simulink model "Lab5_14102026"  (R2019a)
settings: Solver=VariableStepAuto  StartTime=0.0  StopTime=2  RelTol=1e-3  EnableMultiTasking=on
libraries: dspsigops x1
settings Model: Creator=CSE  LastModifiedBy=Admin
settings DataIOCC: ReturnWorkspaceOutputs=off
settings OptimizationCC: LifeSpan=inf
settings DebuggingCC: SFUnexpectedBacktrackingDiag=warning  SFNoUnconditionalDefaultTransitionDiag=warning  ArithmeticOperatorsInVariantConditions=warning
settings SFSimCC: SimUseLocalCustomCode=off
settings RTWCC: RTWUseLocalCustomCode=off
settings CodeAppCC: StateflowObjectComments=on
settings GRTTargetCC: TargetLangStandard=C89/C90 (ANSI)  GeneratePreprocessorConditionals=Disable all
settings ConfigComp: CovMetricSettings=dw  CovHtmlReporting=on  CovSaveCumulativeToWorkspaceVar=on  CovSaveSingleToWorkspaceVar=on  CovExternalEMLEnable=off

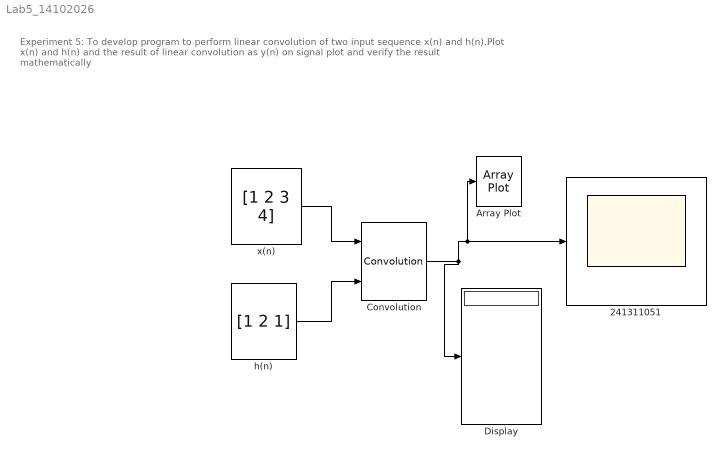
== system Lab5_14102026 ==
  note: Experiment 5: To develop program to perform linear convolution of two input sequence x(n) and h(n).Plot x(n) and h(n) and the result of linear convolution as y(n) on signal plot and verify the result mathematically
  241311051 : Scope
  Array Plot : ArrayPlot
  Convolution : dspsigops/Convolution  domain=Time  roundingMode=Floor  overflowMode=off  outputDataTypeStr=Inherit: Same as accumulator  outputMin=[]  outputMax=[]  outputLastDataTypeStr=Inherit: Same as accumulator
      settings: SourceProductName=DSP System Toolbox  SourceProductBaseCode=DS
  Display : Display
  h(n) : Constant  Value=[1 2 1]  SampleTime=1
  x(n) : Constant  Value=[1 2 3 4]  SampleTime=1
  wires:
  x(n)/1 -> Convolution/1
  h(n)/1 -> Convolution/2
  Convolution/1 -> Array Plot/1, 241311051/1, Display/1
